simulink model "DATA_ADAPTIVE_MODIFIED_PERTURB_AND_OBSERVE_STEADY_STATE_IRRADIATION_VARIATION"  (R2023b)
settings: Solver=ode23  StartTime=0.0  StopTime=0.5  RelTol=1e-7
undefined symbols (not defined in the file): Acid, Lead
libraries: spsMeanLib x40, spsSeriesRLCBranchLib x25, spsVoltageMeasurementLib x20, simulink x10, spsCurrentMeasurementLib x10, spsBatteryLib x5, spsDiodeLib x5, spsMosfetLib x5, spsPVArrayLib x5, spsPWMGeneratorDCDCLib x5, sps_lib x1
(part 2 of 2)

== matlab function DATA_ADAPTIVE_MODIFIED_PERTURB_AND_OBSERVE_STEADY_STATE_IRRADIATION_VARIATION/iradiasi 800/MATLAB Function ==
  data: G input; P_max output; T input
function P_max = Pmax_Teori(G, T)
    % Parameter PV Array Piksel Liar / User-Defined
    P_stc = 10.08;   % Daya Maksimum (Watt)
    G_stc = 1000;    % Iradiasi standar (W/m^2)
    T_stc = 25;      % Suhu standar (Celcius)
    
    % Koefisien suhu untuk daya (dalam desimal)
    gamma = -0.0025899; 
    
    % Perhitungan Daya Maksimum Teoritis Dinamis
    P_max = P_stc * (G/G_stc) * (1 + gamma * (T - T_stc));
end

== matlab function DATA_ADAPTIVE_MODIFIED_PERTURB_AND_OBSERVE_STEADY_STATE_IRRADIATION_VARIATION/iradiasi 600/MATLAB Function ==
  data: G input; P_max output; T input
function P_max = Pmax_Teori(G, T)
    % Parameter PV Array Piksel Liar / User-Defined
    P_stc = 10.08;   % Daya Maksimum (Watt)
    G_stc = 1000;    % Iradiasi standar (W/m^2)
    T_stc = 25;      % Suhu standar (Celcius)
    
    % Koefisien suhu untuk daya (dalam desimal)
    gamma = -0.0025899; 
    
    % Perhitungan Daya Maksimum Teoritis Dinamis
    P_max = P_stc * (G/G_stc) * (1 + gamma * (T - T_stc));
end
